simulink library "xps_library"  (Simulink 8.0)
settings: Solver=ode45  SolverMode=SingleTasking  StartTime=0.0  StopTime=10.0  RelTol=1e-3
undefined symbols (not defined in the file): sys_clk, xps_library_software_register_user_data_in
libraries: xbsIndex_r4 x867, simulink x109, dspsigops x81, casper_library_flow_control x68, xps_library x18, casper_library_misc x11
(part 2 of 10)

== system xps_library/XAUI ==
  rx_get : Inport
  rx_reset : Inport  Port=2
  tx_data : Inport  Port=3
  tx_outofband : Inport  Port=4
  tx_valid : Inport  Port=5
  Constant{1..7} (7 alike) : Constant  Value=0
  Terminator{,1..4} (5 alike) : Terminator
  convert_rx_get : xbsIndex_r4/Convert  gui_display_data_type=Fixed-point  arith_type=Boolean  n_bits=64  bin_pt=0  float_type=Single  exp_bits=8  fraction_bits=24  quantization=Truncate  overflow=Wrap  en=off  latency=0  dbl_ovrd=off  pipeline=off  block_type=convert
      settings: xl_area=[0, 0, 0, 0, 0, 0, 0]
  convert_rx_reset : xbsIndex_r4/Convert  gui_display_data_type=Fixed-point  arith_type=Boolean  n_bits=1  bin_pt=0  float_type=Single  exp_bits=8  fraction_bits=24  quantization=Truncate  overflow=Wrap  en=off  latency=0  dbl_ovrd=off  pipeline=off  block_type=convert
      settings: xl_area=[0, 0, 0, 0, 0, 0, 0]
  convert_tx_data : xbsIndex_r4/Convert  gui_display_data_type=Fixed-point  arith_type=Unsigned  n_bits=64  bin_pt=0  float_type=Single  exp_bits=8  fraction_bits=24  quantization=Truncate  overflow=Wrap  en=off  latency=0  dbl_ovrd=off  pipeline=off  block_type=convert
      settings: xl_area=[0, 0, 0, 0, 0, 0, 0]
  convert_tx_outofband : xbsIndex_r4/Convert  gui_display_data_type=Fixed-point  arith_type=Unsigned  n_bits=8  bin_pt=0  float_type=Single  exp_bits=8  fraction_bits=24  quantization=Truncate  overflow=Wrap  en=off  latency=0  dbl_ovrd=off  pipeline=off  block_type=convert
      settings: xl_area=[0, 0, 0, 0, 0, 0, 0]
  convert_tx_valid : xbsIndex_r4/Convert  gui_display_data_type=Fixed-point  arith_type=Boolean  n_bits=1  bin_pt=0  float_type=Single  exp_bits=8  fraction_bits=24  quantization=Truncate  overflow=Wrap  en=off  latency=0  dbl_ovrd=off  pipeline=off  block_type=convert
      settings: xl_area=[0, 0, 0, 0, 0, 0, 0]
  r_xaui_test_XAUI_rx_almost_full : xbsIndex_r4/Gateway In  gui_display_data_type=Fixed-point  arith_type=Boolean  n_bits=1  bin_pt=0  preci_type=Single  exp_width=8  frac_width=24  quantization=Truncate  overflow=Wrap  period=1  dbl_ovrd=off  timing_constraint=None  locs_specified=off  LOCs={}  hdl_port=on  block_type=gatewayin
      settings: infoedit="Gateway in block.  Converts inputs of type Simulink integer, double and fixed point to  Xilinx fixed point type.<P><P>Hardware notes:  In hardware these blocks become top level input ports."  xl_area=[0, 0, 0, 0, 0, 0, 0]
  r_xaui_test_XAUI_rx_data : xbsIndex_r4/Gateway In  gui_display_data_type=Fixed-point  arith_type=Unsigned  n_bits=64  bin_pt=0  preci_type=Single  exp_width=8  frac_width=24  quantization=Truncate  overflow=Wrap  period=1  dbl_ovrd=off  timing_constraint=None  locs_specified=off  LOCs={}  hdl_port=on  block_type=gatewayin
      settings: infoedit="Gateway in block.  Converts inputs of type Simulink integer, double and fixed point to  Xilinx fixed point type.<P><P>Hardware notes:  In hardware these blocks become top level input ports."  xl_area=[0, 0, 0, 0, 0, 0, 0]
  r_xaui_test_XAUI_rx_empty : xbsIndex_r4/Gateway In  gui_display_data_type=Fixed-point  arith_type=Boolean  n_bits=1  bin_pt=0  preci_type=Single  exp_width=8  frac_width=24  quantization=Truncate  overflow=Wrap  period=1  dbl_ovrd=off  timing_constraint=None  locs_specified=off  LOCs={}  hdl_port=on  block_type=gatewayin
      settings: infoedit="Gateway in block.  Converts inputs of type Simulink integer, double and fixed point to  Xilinx fixed point type.<P><P>Hardware notes:  In hardware these blocks become top level input ports."  xl_area=[0, 0, 0, 0, 0, 0, 0]
  r_xaui_test_XAUI_rx_get : xbsIndex_r4/Gateway Out  hdl_port=on  timing_constraint=None  locs_specified=off  LOCs={}  block_type=gatewayout
      settings: infoedit="Gateway out block.  Converts Xilinx fixed point inputs into ouputs of type Simulink integer, double, or fixed point.<P><P>Hardware notes:  In hardware these blocks become top level output ports or are discarded, depending on how they are configured."  xl_area=[0, 0, 0, 0, 0, 0, 0]
  r_xaui_test_XAUI_rx_linkdown : xbsIndex_r4/Gateway In  gui_display_data_type=Fixed-point  arith_type=Boolean  n_bits=1  bin_pt=0  preci_type=Single  exp_width=8  frac_width=24  quantization=Truncate  overflow=Wrap  period=1  dbl_ovrd=off  timing_constraint=None  locs_specified=off  LOCs={}  hdl_port=on  block_type=gatewayin
      settings: infoedit="Gateway in block.  Converts inputs of type Simulink integer, double and fixed point to  Xilinx fixed point type.<P><P>Hardware notes:  In hardware these blocks become top level input ports."  xl_area=[0, 0, 0, 0, 0, 0, 0]
  r_xaui_test_XAUI_rx_outofband : xbsIndex_r4/Gateway In  gui_display_data_type=Fixed-point  arith_type=Unsigned  n_bits=8  bin_pt=0  preci_type=Single  exp_width=8  frac_width=24  quantization=Truncate  overflow=Wrap  period=1  dbl_ovrd=off  timing_constraint=None  locs_specified=off  LOCs={}  hdl_port=on  block_type=gatewayin
      settings: infoedit="Gateway in block.  Converts inputs of type Simulink integer, double and fixed point to  Xilinx fixed point type.<P><P>Hardware notes:  In hardware these blocks become top level input ports."  xl_area=[0, 0, 0, 0, 0, 0, 0]
  r_xaui_test_XAUI_rx_reset : xbsIndex_r4/Gateway Out  hdl_port=on  timing_constraint=None  locs_specified=off  LOCs={}  block_type=gatewayout
      settings: infoedit="Gateway out block.  Converts Xilinx fixed point inputs into ouputs of type Simulink integer, double, or fixed point.<P><P>Hardware notes:  In hardware these blocks become top level output ports or are discarded, depending on how they are configured."  xl_area=[0, 0, 0, 0, 0, 0, 0]
  r_xaui_test_XAUI_rx_valid : xbsIndex_r4/Gateway In  gui_display_data_type=Fixed-point  arith_type=Boolean  n_bits=1  bin_pt=0  preci_type=Single  exp_width=8  frac_width=24  quantization=Truncate  overflow=Wrap  period=1  dbl_ovrd=off  timing_constraint=None  locs_specified=off  LOCs={}  hdl_port=on  block_type=gatewayin
      settings: infoedit="Gateway in block.  Converts inputs of type Simulink integer, double and fixed point to  Xilinx fixed point type.<P><P>Hardware notes:  In hardware these blocks become top level input ports."  xl_area=[0, 0, 0, 0, 0, 0, 0]
  r_xaui_test_XAUI_tx_data : xbsIndex_r4/Gateway Out  hdl_port=on  timing_constraint=None  locs_specified=off  LOCs={}  block_type=gatewayout
      settings: infoedit="Gateway out block.  Converts Xilinx fixed point inputs into ouputs of type Simulink integer, double, or fixed point.<P><P>Hardware notes:  In hardware these blocks become top level output ports or are discarded, depending on how they are configured."  xl_area=[0, 0, 0, 0, 0, 0, 0]
  r_xaui_test_XAUI_tx_full : xbsIndex_r4/Gateway In  gui_display_data_type=Fixed-point  arith_type=Boolean  n_bits=1  bin_pt=0  preci_type=Single  exp_width=8  frac_width=24  quantization=Truncate  overflow=Wrap  period=1  dbl_ovrd=off  timing_constraint=None  locs_specified=off  LOCs={}  hdl_port=on  block_type=gatewayin
      settings: infoedit="Gateway in block.  Converts inputs of type Simulink integer, double and fixed point to  Xilinx fixed point type.<P><P>Hardware notes:  In hardware these blocks become top level input ports."  xl_area=[0, 0, 0, 0, 0, 0, 0]
  r_xaui_test_XAUI_tx_outofband : xbsIndex_r4/Gateway Out  hdl_port=on  timing_constraint=None  locs_specified=off  LOCs={}  block_type=gatewayout
      settings: infoedit="Gateway out block.  Converts Xilinx fixed point inputs into ouputs of type Simulink integer, double, or fixed point.<P><P>Hardware notes:  In hardware these blocks become top level output ports or are discarded, depending on how they are configured."  xl_area=[0, 0, 0, 0, 0, 0, 0]
  r_xaui_test_XAUI_tx_valid : xbsIndex_r4/Gateway Out  hdl_port=on  timing_constraint=None  locs_specified=off  LOCs={}  block_type=gatewayout
      settings: infoedit="Gateway out block.  Converts Xilinx fixed point inputs into ouputs of type Simulink integer, double, or fixed point.<P><P>Hardware notes:  In hardware these blocks become top level output ports or are discarded, depending on how they are configured."  xl_area=[0, 0, 0, 0, 0, 0, 0]
  rx_data : Outport
  rx_outofband : Outport  Port=2
  rx_empty : Outport  Port=3
  rx_valid : Outport  Port=4
  rx_linkdown : Outport  Port=5
  tx_full : Outport  Port=6
  rx_almost_full : Outport  Port=7
  wires:
  rx_get/1 -> convert_rx_get/1
  convert_rx_get/1 -> r_xaui_test_XAUI_rx_get/1
  rx_reset/1 -> convert_rx_reset/1
  convert_rx_reset/1 -> r_xaui_test_XAUI_rx_reset/1
  r_xaui_test_XAUI_rx_data/1 -> rx_data/1
  r_xaui_test_XAUI_rx_outofband/1 -> rx_outofband/1
  r_xaui_test_XAUI_rx_empty/1 -> rx_empty/1
  r_xaui_test_XAUI_rx_linkdown/1 -> rx_linkdown/1
  tx_data/1 -> convert_tx_data/1
  convert_tx_data/1 -> r_xaui_test_XAUI_tx_data/1
  tx_outofband/1 -> convert_tx_outofband/1
  convert_tx_outofband/1 -> r_xaui_test_XAUI_tx_outofband/1
  tx_valid/1 -> convert_tx_valid/1
  convert_tx_valid/1 -> r_xaui_test_XAUI_tx_valid/1
  r_xaui_test_XAUI_tx_full/1 -> tx_full/1
  r_xaui_test_XAUI_tx_data/1 -> Terminator/1
  r_xaui_test_XAUI_tx_outofband/1 -> Terminator1/1
  r_xaui_test_XAUI_tx_valid/1 -> Terminator2/1
  Constant2/1 -> r_xaui_test_XAUI_tx_full/1
  Constant3/1 -> r_xaui_test_XAUI_rx_linkdown/1
  Constant4/1 -> r_xaui_test_XAUI_rx_empty/1
  Constant5/1 -> r_xaui_test_XAUI_rx_outofband/1
  Constant6/1 -> r_xaui_test_XAUI_rx_data/1
  r_xaui_test_XAUI_rx_get/1 -> Terminator3/1
  r_xaui_test_XAUI_rx_reset/1 -> Terminator4/1
  Constant7/1 -> r_xaui_test_XAUI_rx_valid/1
  r_xaui_test_XAUI_rx_valid/1 -> rx_valid/1
  r_xaui_test_XAUI_rx_almost_full/1 -> rx_almost_full/1
  Constant1/1 -> r_xaui_test_XAUI_rx_almost_full/1

== system xps_library/XSG core config ==

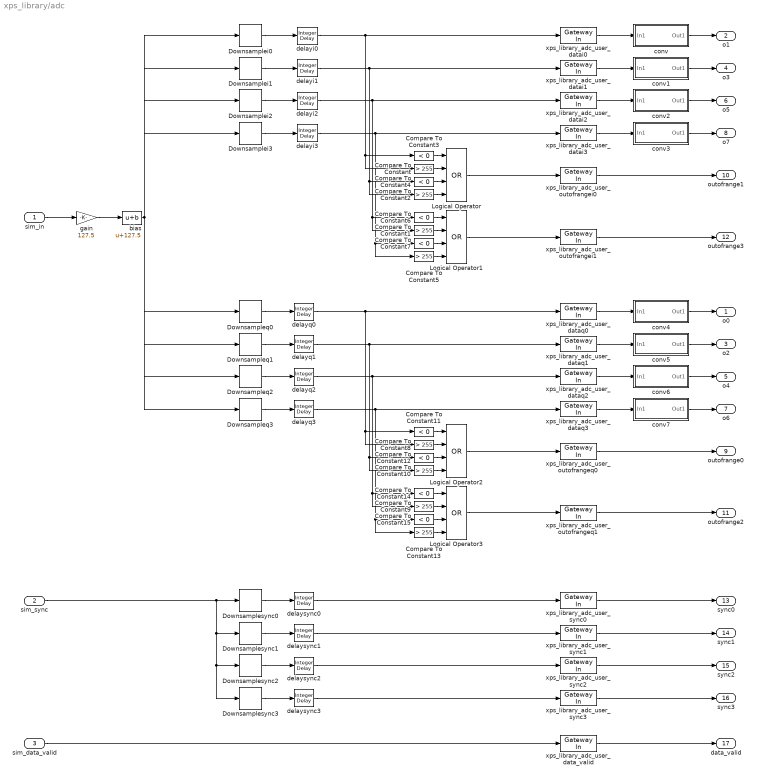
== system xps_library/adc ==
  sim_in : Inport  SampleTime=sample_period/8
  sim_sync : Inport  Port=2  SampleTime=sample_period/8
  sim_data_valid : Inport  Port=3  SampleTime=sample_period/4
  Compare To Constant{,1..2,5,8..10,13} (8 alike) : simulink/Logic and Bit Operations/Compare To Constant  relop=>  const=255  LogicOutDataTypeMode=boolean  ZeroCross=off
  Compare To Constant{3..4,6..7,11..12,14..15} (8 alike) : simulink/Logic and Bit Operations/Compare To Constant  relop=<  const=0  LogicOutDataTypeMode=boolean  ZeroCross=off
  Downsamplei0 : dspsigops/Downsample  N=8  phase=1  smode=Allow multirate  fmode=Maintain input frame size  ic=0
  Downsamplei1 : dspsigops/Downsample  N=8  phase=3  smode=Allow multirate  fmode=Maintain input frame size  ic=0
  Downsamplei2 : dspsigops/Downsample  N=8  phase=5  smode=Allow multirate  fmode=Maintain input frame size  ic=0
  Downsamplei3 : dspsigops/Downsample  N=8  phase=7  smode=Allow multirate  fmode=Maintain input frame size  ic=0
  Downsampleq0 : dspsigops/Downsample  N=8  phase=0  smode=Allow multirate  fmode=Maintain input frame size  ic=0
  Downsampleq1 : dspsigops/Downsample  N=8  phase=2  smode=Allow multirate  fmode=Maintain input frame size  ic=0
  Downsampleq2 : dspsigops/Downsample  N=8  phase=4  smode=Allow multirate  fmode=Maintain input frame size  ic=0
  Downsampleq3 : dspsigops/Downsample  N=8  phase=6  smode=Allow multirate  fmode=Maintain input frame size  ic=0
  Downsamplesync0 : dspsigops/Downsample  N=8  phase=0  smode=Allow multirate  fmode=Maintain input frame size  ic=0
  Downsamplesync1 : dspsigops/Downsample  N=8  phase=2  smode=Allow multirate  fmode=Maintain input frame size  ic=0
  Downsamplesync2 : dspsigops/Downsample  N=8  phase=4  smode=Allow multirate  fmode=Maintain input frame size  ic=0
  Downsamplesync3 : dspsigops/Downsample  N=8  phase=6  smode=Allow multirate  fmode=Maintain input frame size  ic=0
  Logical Operator{,1..3} (4 alike) : Logic  Operator=OR  Inputs=4  AllPortsSameDT=off  OutDataTypeStr=boolean
  bias : Bias  Bias=127.5  SaturateOnIntegerOverflow=on
  conv : Subsystem
  conv1 : Subsystem
  conv2 : Subsystem
  conv3 : Subsystem
  conv4 : Subsystem
  conv5 : Subsystem
  conv6 : Subsystem
  conv7 : Subsystem
  delayi{0..3} (4 alike) : simulink/Discrete/Integer Delay  NumDelays=1  vinit=0.0  samptime=-1
  delayq0 : simulink/Discrete/Integer Delay  NumDelays=2  vinit=0.0  samptime=-1
  delayq1 : simulink/Discrete/Integer Delay  NumDelays=1  vinit=0.0  samptime=-1
  delayq2 : simulink/Discrete/Integer Delay  NumDelays=1  vinit=0.0  samptime=-1
  delayq3 : simulink/Discrete/Integer Delay  NumDelays=1  vinit=0.0  samptime=-1
  delaysync0 : simulink/Discrete/Integer Delay  NumDelays=2  vinit=0.0  samptime=-1
  delaysync1 : simulink/Discrete/Integer Delay  NumDelays=1  vinit=0.0  samptime=-1
  delaysync2 : simulink/Discrete/Integer Delay  NumDelays=1  vinit=0.0  samptime=-1
  delaysync3 : simulink/Discrete/Integer Delay  NumDelays=1  vinit=0.0  samptime=-1
  gain : Gain  Gain=127.5  SaturateOnIntegerOverflow=on  OutDataTypeStr=Inherit: Same as input  ParamDataTypeStr=Inherit: Same as input
  xps_library_adc_user_data_valid : xbsIndex_r4/Gateway In  gui_display_data_type=Fixed-point  arith_type=Boolean  n_bits=8  bin_pt=0  preci_type=Single  exp_width=8  frac_width=24  quantization="Round  (unbiased: +/- Inf)"  overflow=Saturate  period=sample_period  dbl_ovrd=off  timing_constraint=None  locs_specified=off  LOCs={}  hdl_port=on  block_type=gatewayin
      settings: infoedit="Gateway in block.  Converts inputs of type Simulink integer, double and fixed point to  Xilinx fixed point type.<P><P>Hardware notes:  In hardware these blocks become top level input ports."  xl_area=[0 0 0 0 8 0 0]  block_version=8.2.02
  xps_library_adc_user_datai{0..3} (4 alike) : xbsIndex_r4/Gateway In  gui_display_data_type=Fixed-point  arith_type=Unsigned  n_bits=8  bin_pt=0  preci_type=Single  exp_width=8  frac_width=24  quantization="Round  (unbiased: +/- Inf)"  overflow=Saturate  period=sample_period  dbl_ovrd=off  timing_constraint=None  locs_specified=off  LOCs={}  hdl_port=on  block_type=gatewayin
      settings: infoedit="Gateway in block.  Converts inputs of type Simulink integer, double and fixed point to  Xilinx fixed point type.<P><P>Hardware notes:  In hardware these blocks become top level input ports."  xl_area=[0 0 0 0 8 0 0]  block_version=8.2.02
  xps_library_adc_user_dataq{0..3} (4 alike) : xbsIndex_r4/Gateway In  gui_display_data_type=Fixed-point  arith_type=Unsigned  n_bits=8  bin_pt=0  preci_type=Single  exp_width=8  frac_width=24  quantization="Round  (unbiased: +/- Inf)"  overflow=Saturate  period=sample_period  dbl_ovrd=off  timing_constraint=None  locs_specified=off  LOCs={}  hdl_port=on  block_type=gatewayin
      settings: infoedit="Gateway in block.  Converts inputs of type Simulink integer, double and fixed point to  Xilinx fixed point type.<P><P>Hardware notes:  In hardware these blocks become top level input ports."  xl_area=[0 0 0 0 8 0 0]  block_version=8.2.02
  xps_library_adc_user_outofrangei0 : xbsIndex_r4/Gateway In  gui_display_data_type=Fixed-point  arith_type=Boolean  n_bits=8  bin_pt=0  preci_type=Single  exp_width=8  frac_width=24  quantization="Round  (unbiased: +/- Inf)"  overflow=Saturate  period=sample_period  dbl_ovrd=off  timing_constraint=None  locs_specified=off  LOCs={}  hdl_port=on  block_type=gatewayin
      settings: infoedit="Gateway in block.  Converts inputs of type Simulink integer, double and fixed point to  Xilinx fixed point type.<P><P>Hardware notes:  In hardware these blocks become top level input ports."  xl_area=[0 0 0 0 8 0 0]  block_version=8.2.02
  xps_library_adc_user_outofrangei1 : xbsIndex_r4/Gateway In  gui_display_data_type=Fixed-point  arith_type=Boolean  n_bits=8  bin_pt=0  preci_type=Single  exp_width=8  frac_width=24  quantization="Round  (unbiased: +/- Inf)"  overflow=Saturate  period=sample_period  dbl_ovrd=off  timing_constraint=None  locs_specified=off  LOCs={}  hdl_port=on  block_type=gatewayin
      settings: infoedit="Gateway in block.  Converts inputs of type Simulink integer, double and fixed point to  Xilinx fixed point type.<P><P>Hardware notes:  In hardware these blocks become top level input ports."  xl_area=[0 0 0 0 8 0 0]  block_version=8.2.02
  xps_library_adc_user_outofrangeq0 : xbsIndex_r4/Gateway In  gui_display_data_type=Fixed-point  arith_type=Boolean  n_bits=8  bin_pt=0  preci_type=Single  exp_width=8  frac_width=24  quantization="Round  (unbiased: +/- Inf)"  overflow=Saturate  period=sample_period  dbl_ovrd=off  timing_constraint=None  locs_specified=off  LOCs={}  hdl_port=on  block_type=gatewayin
      settings: infoedit="Gateway in block.  Converts inputs of type Simulink integer, double and fixed point to  Xilinx fixed point type.<P><P>Hardware notes:  In hardware these blocks become top level input ports."  xl_area=[0 0 0 0 8 0 0]  block_version=8.2.02
  xps_library_adc_user_outofrangeq1 : xbsIndex_r4/Gateway In  gui_display_data_type=Fixed-point  arith_type=Boolean  n_bits=8  bin_pt=0  preci_type=Single  exp_width=8  frac_width=24  quantization="Round  (unbiased: +/- Inf)"  overflow=Saturate  period=sample_period  dbl_ovrd=off  timing_constraint=None  locs_specified=off  LOCs={}  hdl_port=on  block_type=gatewayin
      settings: infoedit="Gateway in block.  Converts inputs of type Simulink integer, double and fixed point to  Xilinx fixed point type.<P><P>Hardware notes:  In hardware these blocks become top level input ports."  xl_area=[0 0 0 0 8 0 0]  block_version=8.2.02
  xps_library_adc_user_sync{0..3} (4 alike) : xbsIndex_r4/Gateway In  gui_display_data_type=Fixed-point  arith_type=Boolean  n_bits=8  bin_pt=0  preci_type=Single  exp_width=8  frac_width=24  quantization="Round  (unbiased: +/- Inf)"  overflow=Saturate  period=sample_period  dbl_ovrd=off  timing_constraint=None  locs_specified=off  LOCs={}  hdl_port=on  block_type=gatewayin
      settings: infoedit="Gateway in block.  Converts inputs of type Simulink integer, double and fixed point to  Xilinx fixed point type.<P><P>Hardware notes:  In hardware these blocks become top level input ports."  xl_area=[0 0 0 0 8 0 0]  block_version=8.2.02
  o0 : Outport
  o1 : Outport  Port=2
  o2 : Outport  Port=3
  o3 : Outport  Port=4
  o4 : Outport  Port=5
  o5 : Outport  Port=6
  o6 : Outport  Port=7
  o7 : Outport  Port=8
  outofrange0 : Outport  Port=9
  outofrange1 : Outport  Port=10
  outofrange2 : Outport  Port=11
  outofrange3 : Outport  Port=12
  sync0 : Outport  Port=13
  sync1 : Outport  Port=14
  sync2 : Outport  Port=15
  sync3 : Outport  Port=16
  data_valid : Outport  Port=17
  wires:
  delaysync1/1 -> xps_library_adc_user_sync1/1
  delayq3/1 -> xps_library_adc_user_dataq3/1, Compare To Constant15/1, Compare To Constant13/1
  delayq2/1 -> xps_library_adc_user_dataq2/1, Compare To Constant14/1, Compare To Constant9/1
  delayq1/1 -> xps_library_adc_user_dataq1/1, Compare To Constant12/1, Compare To Constant10/1
  delayi3/1 -> xps_library_adc_user_datai3/1, Compare To Constant7/1, Compare To Constant5/1
  delayi2/1 -> xps_library_adc_user_datai2/1, Compare To Constant6/1, Compare To Constant1/1
  delayi1/1 -> xps_library_adc_user_datai1/1, Compare To Constant2/1, Compare To Constant4/1
  Downsamplei0/1 -> delayi0/1
  conv7/1(Out1) -> o6/1
  xps_library_adc_user_dataq3/1 -> conv7/1(In1)
  conv6/1(Out1) -> o4/1
  xps_library_adc_user_dataq2/1 -> conv6/1(In1)
  conv5/1(Out1) -> o2/1
  xps_library_adc_user_dataq1/1 -> conv5/1(In1)
  conv4/1(Out1) -> o0/1
  xps_library_adc_user_dataq0/1 -> conv4/1(In1)
  conv3/1(Out1) -> o7/1
  conv2/1(Out1) -> o5/1
  conv1/1(Out1) -> o3/1
  conv/1(Out1) -> o1/1
  xps_library_adc_user_sync0/1 -> sync0/1
  xps_library_adc_user_outofrangei0/1 -> outofrange1/1
  xps_library_adc_user_datai3/1 -> conv3/1(In1)
  xps_library_adc_user_datai2/1 -> conv2/1(In1)
  xps_library_adc_user_datai1/1 -> conv1/1(In1)
  Downsampleq3/1 -> delayq3/1
  Downsampleq2/1 -> delayq2/1
  Downsampleq1/1 -> delayq1/1
  Downsamplei3/1 -> delayi3/1
  Downsamplei2/1 -> delayi2/1
  Downsamplei1/1 -> delayi1/1
  delayi0/1 -> xps_library_adc_user_datai0/1, Compare To Constant/1, Compare To Constant3/1
  Downsampleq0/1 -> delayq0/1
  delayq0/1 -> xps_library_adc_user_dataq0/1, Compare To Constant11/1, Compare To Constant8/1
  xps_library_adc_user_outofrangei1/1 -> outofrange3/1
  Compare To Constant3/1 -> Logical Operator/1
  Compare To Constant/1 -> Logical Operator/2
  Compare To Constant4/1 -> Logical Operator/3
  Compare To Constant2/1 -> Logical Operator/4
  Logical Operator/1 -> xps_library_adc_user_outofrangei0/1
  Compare To Constant6/1 -> Logical Operator1/1
  Compare To Constant1/1 -> Logical Operator1/2
  Compare To Constant7/1 -> Logical Operator1/3
  Compare To Constant5/1 -> Logical Operator1/4
  Logical Operator1/1 -> xps_library_adc_user_outofrangei1/1
  xps_library_adc_user_outofrangeq0/1 -> outofrange0/1
  xps_library_adc_user_outofrangeq1/1 -> outofrange2/1
  Compare To Constant11/1 -> Logical Operator2/1
  Compare To Constant8/1 -> Logical Operator2/2
  Compare To Constant12/1 -> Logical Operator2/3
  Compare To Constant10/1 -> Logical Operator2/4
  Logical Operator2/1 -> xps_library_adc_user_outofrangeq0/1
  Compare To Constant14/1 -> Logical Operator3/1
  Compare To Constant9/1 -> Logical Operator3/2
  Compare To Constant15/1 -> Logical Operator3/3
  Compare To Constant13/1 -> Logical Operator3/4
  Logical Operator3/1 -> xps_library_adc_user_outofrangeq1/1
  sim_sync/1 -> Downsamplesync0/1, Downsamplesync1/1, Downsamplesync2/1, Downsamplesync3/1
  Downsamplesync0/1 -> delaysync0/1
  Downsamplesync1/1 -> delaysync1/1
  delaysync0/1 -> xps_library_adc_user_sync0/1
  xps_library_adc_user_sync1/1 -> sync1/1
  Downsamplesync2/1 -> delaysync2/1
  Downsamplesync3/1 -> delaysync3/1
  delaysync2/1 -> xps_library_adc_user_sync2/1
  delaysync3/1 -> xps_library_adc_user_sync3/1
  xps_library_adc_user_sync2/1 -> sync2/1
  xps_library_adc_user_sync3/1 -> sync3/1
  xps_library_adc_user_data_valid/1 -> data_valid/1
  sim_data_valid/1 -> xps_library_adc_user_data_valid/1
  xps_library_adc_user_datai0/1 -> conv/1(In1)
  sim_in/1 -> gain/1
  gain/1 -> bias/1
  bias/1 -> Downsamplei0/1, Downsamplei1/1, Downsamplei2/1, Downsamplei3/1, Downsampleq0/1, Downsampleq1/1, Downsampleq2/1, Downsampleq3/1

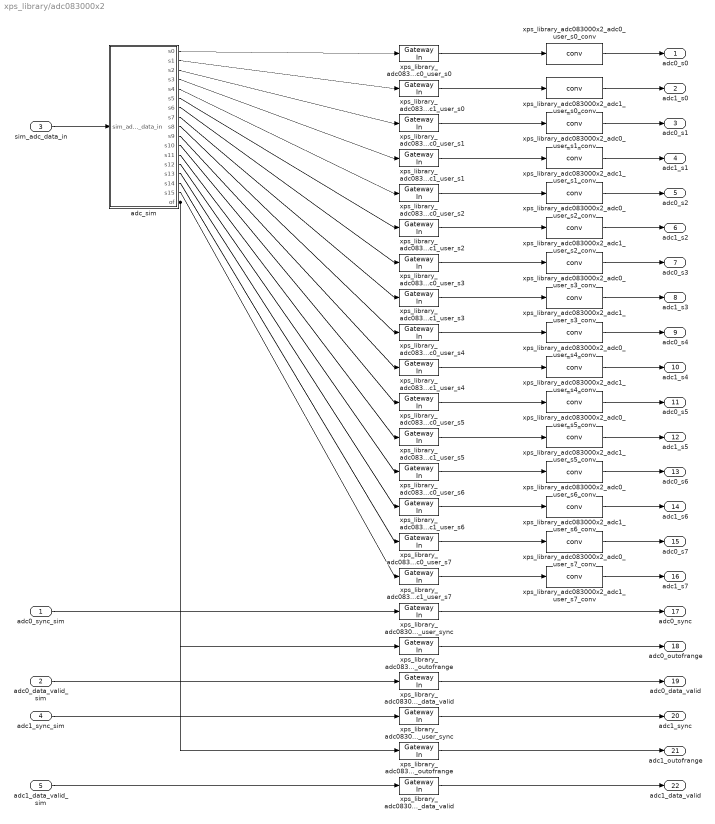
== system xps_library/adc083000x2 ==
  adc0_sync_sim : Inport
  adc0_data_valid_sim : Inport  Port=2
  sim_adc_data_in : Inport  Port=3
  adc1_sync_sim : Inport  Port=4
  adc1_data_valid_sim : Inport  Port=5
  adc_sim : Subsystem  AncestorBlock=xps_library/ADCs/adc_sim  mask(adc_sim){nStreams=16, bit_width=8}
      mask prompts: nStreams "Number of Output Streams"; bit_width "Sample Bit Width"
      mask help:
      | This block simulates the behavior of a demuxed ADC, which takes
      | as input a waveform and returns digital samples in parallel at
      | a slower rate.
      |
      | This block is used to simulate the behavior
      mask init:
      | adc_sim_init(gcb, ...
      |     'nStreams', nStreams, ...
      |     'bit_width', bit_width);
  xps_library_adc083000x2_adc0_user_data_valid : xbsIndex_r4/Gateway In  gui_display_data_type=Fixed-point  arith_type=Unsigned  n_bits=1  bin_pt=0  preci_type=Single  exp_width=8  frac_width=24  quantization="Round  (unbiased: +/- Inf)"  overflow=Saturate  period=1  dbl_ovrd=off  timing_constraint=None  locs_specified=off  LOCs={}  hdl_port=on  block_type=gatewayin
  xps_library_adc083000x2_adc0_user_outofrange : xbsIndex_r4/Gateway In  gui_display_data_type=Fixed-point  arith_type=Unsigned  n_bits=4  bin_pt=0  preci_type=Single  exp_width=8  frac_width=24  quantization="Round  (unbiased: +/- Inf)"  overflow=Saturate  period=1  dbl_ovrd=off  timing_constraint=None  locs_specified=off  LOCs={}  hdl_port=on  block_type=gatewayin
  xps_library_adc083000x2_adc0_user_s{0..7} (8 alike) : xbsIndex_r4/Gateway In  gui_display_data_type=Fixed-point  arith_type=Unsigned  n_bits=8  bin_pt=0  preci_type=Single  exp_width=8  frac_width=24  quantization="Round  (unbiased: +/- Inf)"  overflow=Saturate  period=1  dbl_ovrd=off  timing_constraint=None  locs_specified=off  LOCs={}  hdl_port=on  block_type=gatewayin
  xps_library_adc083000x2_adc0_user_s0_conv : xps_library/ADCs/conv  bit_width=8
  xps_library_adc083000x2_adc0_user_s1_conv : xps_library/ADCs/conv  bit_width=8
  xps_library_adc083000x2_adc0_user_s2_conv : xps_library/ADCs/conv  bit_width=8
  xps_library_adc083000x2_adc0_user_s3_conv : xps_library/ADCs/conv  bit_width=8
  xps_library_adc083000x2_adc0_user_s4_conv : xps_library/ADCs/conv  bit_width=8
  xps_library_adc083000x2_adc0_user_s5_conv : xps_library/ADCs/conv  bit_width=8
  xps_library_adc083000x2_adc0_user_s6_conv : xps_library/ADCs/conv  bit_width=8
  xps_library_adc083000x2_adc0_user_s7_conv : xps_library/ADCs/conv  bit_width=8
  xps_library_adc083000x2_adc0_user_sync : xbsIndex_r4/Gateway In  gui_display_data_type=Fixed-point  arith_type=Unsigned  n_bits=4  bin_pt=0  preci_type=Single  exp_width=8  frac_width=24  quantization="Round  (unbiased: +/- Inf)"  overflow=Saturate  period=1  dbl_ovrd=off  timing_constraint=None  locs_specified=off  LOCs={}  hdl_port=on  block_type=gatewayin
  xps_library_adc083000x2_adc1_user_data_valid : xbsIndex_r4/Gateway In  gui_display_data_type=Fixed-point  arith_type=Unsigned  n_bits=1  bin_pt=0  preci_type=Single  exp_width=8  frac_width=24  quantization="Round  (unbiased: +/- Inf)"  overflow=Saturate  period=1  dbl_ovrd=off  timing_constraint=None  locs_specified=off  LOCs={}  hdl_port=on  block_type=gatewayin  OutDataTypeMode=boolean
  xps_library_adc083000x2_adc1_user_outofrange : xbsIndex_r4/Gateway In  gui_display_data_type=Fixed-point  arith_type=Unsigned  n_bits=4  bin_pt=0  preci_type=Single  exp_width=8  frac_width=24  quantization="Round  (unbiased: +/- Inf)"  overflow=Saturate  period=1  dbl_ovrd=off  timing_constraint=None  locs_specified=off  LOCs={}  hdl_port=on  block_type=gatewayin
  xps_library_adc083000x2_adc1_user_s{0..7} (8 alike) : xbsIndex_r4/Gateway In  gui_display_data_type=Fixed-point  arith_type=Unsigned  n_bits=8  bin_pt=0  preci_type=Single  exp_width=8  frac_width=24  quantization="Round  (unbiased: +/- Inf)"  overflow=Saturate  period=1  dbl_ovrd=off  timing_constraint=None  locs_specified=off  LOCs={}  hdl_port=on  block_type=gatewayin
  xps_library_adc083000x2_adc1_user_s0_conv : xps_library/ADCs/conv  bit_width=8
  xps_library_adc083000x2_adc1_user_s1_conv : xps_library/ADCs/conv  bit_width=8
  xps_library_adc083000x2_adc1_user_s2_conv : xps_library/ADCs/conv  bit_width=8
  xps_library_adc083000x2_adc1_user_s3_conv : xps_library/ADCs/conv  bit_width=8
  xps_library_adc083000x2_adc1_user_s4_conv : xps_library/ADCs/conv  bit_width=8
  xps_library_adc083000x2_adc1_user_s5_conv : xps_library/ADCs/conv  bit_width=8
  xps_library_adc083000x2_adc1_user_s6_conv : xps_library/ADCs/conv  bit_width=8
  xps_library_adc083000x2_adc1_user_s7_conv : xps_library/ADCs/conv  bit_width=8
  xps_library_adc083000x2_adc1_user_sync : xbsIndex_r4/Gateway In  gui_display_data_type=Fixed-point  arith_type=Unsigned  n_bits=4  bin_pt=0  preci_type=Single  exp_width=8  frac_width=24  quantization="Round  (unbiased: +/- Inf)"  overflow=Saturate  period=1  dbl_ovrd=off  timing_constraint=None  locs_specified=off  LOCs={}  hdl_port=on  block_type=gatewayin
  adc0_s0 : Outport
  adc1_s0 : Outport  Port=2
  adc0_s1 : Outport  Port=3
  adc1_s1 : Outport  Port=4
  adc0_s2 : Outport  Port=5
  adc1_s2 : Outport  Port=6
  adc0_s3 : Outport  Port=7
  adc1_s3 : Outport  Port=8
  adc0_s4 : Outport  Port=9
  adc1_s4 : Outport  Port=10
  adc0_s5 : Outport  Port=11
  adc1_s5 : Outport  Port=12
  adc0_s6 : Outport  Port=13
  adc1_s6 : Outport  Port=14
  adc0_s7 : Outport  Port=15
  adc1_s7 : Outport  Port=16
  adc0_sync : Outport  Port=17
  adc0_outofrange : Outport  Port=18
  adc0_data_valid : Outport  Port=19
  adc1_sync : Outport  Port=20
  adc1_outofrange : Outport  Port=21
  adc1_data_valid : Outport  Port=22
  wires:
  sim_adc_data_in/1 -> adc_sim/1(sim_adc_data_in)
  adc_sim/1(s0) -> xps_library_adc083000x2_adc0_user_s0/1
  xps_library_adc083000x2_adc0_user_s0/1 -> xps_library_adc083000x2_adc0_user_s0_conv/1
  xps_library_adc083000x2_adc0_user_s0_conv/1 -> adc0_s0/1
  adc_sim/2(s1) -> xps_library_adc083000x2_adc1_user_s0/1
  xps_library_adc083000x2_adc1_user_s0/1 -> xps_library_adc083000x2_adc1_user_s0_conv/1
  xps_library_adc083000x2_adc1_user_s0_conv/1 -> adc1_s0/1
  adc_sim/3(s2) -> xps_library_adc083000x2_adc0_user_s1/1
  xps_library_adc083000x2_adc0_user_s1/1 -> xps_library_adc083000x2_adc0_user_s1_conv/1
  xps_library_adc083000x2_adc0_user_s1_conv/1 -> adc0_s1/1
  adc_sim/4(s3) -> xps_library_adc083000x2_adc1_user_s1/1
  xps_library_adc083000x2_adc1_user_s1/1 -> xps_library_adc083000x2_adc1_user_s1_conv/1
  xps_library_adc083000x2_adc1_user_s1_conv/1 -> adc1_s1/1
  adc_sim/5(s4) -> xps_library_adc083000x2_adc0_user_s2/1
  xps_library_adc083000x2_adc0_user_s2/1 -> xps_library_adc083000x2_adc0_user_s2_conv/1
  xps_library_adc083000x2_adc0_user_s2_conv/1 -> adc0_s2/1
  adc_sim/6(s5) -> xps_library_adc083000x2_adc1_user_s2/1
  xps_library_adc083000x2_adc1_user_s2/1 -> xps_library_adc083000x2_adc1_user_s2_conv/1
  xps_library_adc083000x2_adc1_user_s2_conv/1 -> adc1_s2/1
  adc_sim/7(s6) -> xps_library_adc083000x2_adc0_user_s3/1
  xps_library_adc083000x2_adc0_user_s3/1 -> xps_library_adc083000x2_adc0_user_s3_conv/1
  xps_library_adc083000x2_adc0_user_s3_conv/1 -> adc0_s3/1
  adc_sim/8(s7) -> xps_library_adc083000x2_adc1_user_s3/1
  xps_library_adc083000x2_adc1_user_s3/1 -> xps_library_adc083000x2_adc1_user_s3_conv/1
  xps_library_adc083000x2_adc1_user_s3_conv/1 -> adc1_s3/1
  adc_sim/9(s8) -> xps_library_adc083000x2_adc0_user_s4/1
  xps_library_adc083000x2_adc0_user_s4/1 -> xps_library_adc083000x2_adc0_user_s4_conv/1
  xps_library_adc083000x2_adc0_user_s4_conv/1 -> adc0_s4/1
  adc_sim/10(s9) -> xps_library_adc083000x2_adc1_user_s4/1
  xps_library_adc083000x2_adc1_user_s4/1 -> xps_library_adc083000x2_adc1_user_s4_conv/1
  xps_library_adc083000x2_adc1_user_s4_conv/1 -> adc1_s4/1
  adc_sim/11(s10) -> xps_library_adc083000x2_adc0_user_s5/1
  xps_library_adc083000x2_adc0_user_s5/1 -> xps_library_adc083000x2_adc0_user_s5_conv/1
  xps_library_adc083000x2_adc0_user_s5_conv/1 -> adc0_s5/1
  adc_sim/12(s11) -> xps_library_adc083000x2_adc1_user_s5/1
  xps_library_adc083000x2_adc1_user_s5/1 -> xps_library_adc083000x2_adc1_user_s5_conv/1
  xps_library_adc083000x2_adc1_user_s5_conv/1 -> adc1_s5/1
  adc_sim/13(s12) -> xps_library_adc083000x2_adc0_user_s6/1
  xps_library_adc083000x2_adc0_user_s6/1 -> xps_library_adc083000x2_adc0_user_s6_conv/1
  xps_library_adc083000x2_adc0_user_s6_conv/1 -> adc0_s6/1
  adc_sim/14(s13) -> xps_library_adc083000x2_adc1_user_s6/1
  xps_library_adc083000x2_adc1_user_s6/1 -> xps_library_adc083000x2_adc1_user_s6_conv/1
  xps_library_adc083000x2_adc1_user_s6_conv/1 -> adc1_s6/1
  adc_sim/15(s14) -> xps_library_adc083000x2_adc0_user_s7/1
  xps_library_adc083000x2_adc0_user_s7/1 -> xps_library_adc083000x2_adc0_user_s7_conv/1
  xps_library_adc083000x2_adc0_user_s7_conv/1 -> adc0_s7/1
  adc_sim/16(s15) -> xps_library_adc083000x2_adc1_user_s7/1
  xps_library_adc083000x2_adc1_user_s7/1 -> xps_library_adc083000x2_adc1_user_s7_conv/1
  xps_library_adc083000x2_adc1_user_s7_conv/1 -> adc1_s7/1
  adc0_sync_sim/1 -> xps_library_adc083000x2_adc0_user_sync/1
  xps_library_adc083000x2_adc0_user_sync/1 -> adc0_sync/1
  adc_sim/17(of) -> xps_library_adc083000x2_adc0_user_outofrange/1, xps_library_adc083000x2_adc1_user_outofrange/1
  xps_library_adc083000x2_adc0_user_outofrange/1 -> adc0_outofrange/1
  adc0_data_valid_sim/1 -> xps_library_adc083000x2_adc0_user_data_valid/1
  xps_library_adc083000x2_adc0_user_data_valid/1 -> adc0_data_valid/1
  adc1_sync_sim/1 -> xps_library_adc083000x2_adc1_user_sync/1
  xps_library_adc083000x2_adc1_user_sync/1 -> adc1_sync/1
  xps_library_adc083000x2_adc1_user_outofrange/1 -> adc1_outofrange/1
  adc1_data_valid_sim/1 -> xps_library_adc083000x2_adc1_user_data_valid/1
  xps_library_adc083000x2_adc1_user_data_valid/1 -> adc1_data_valid/1

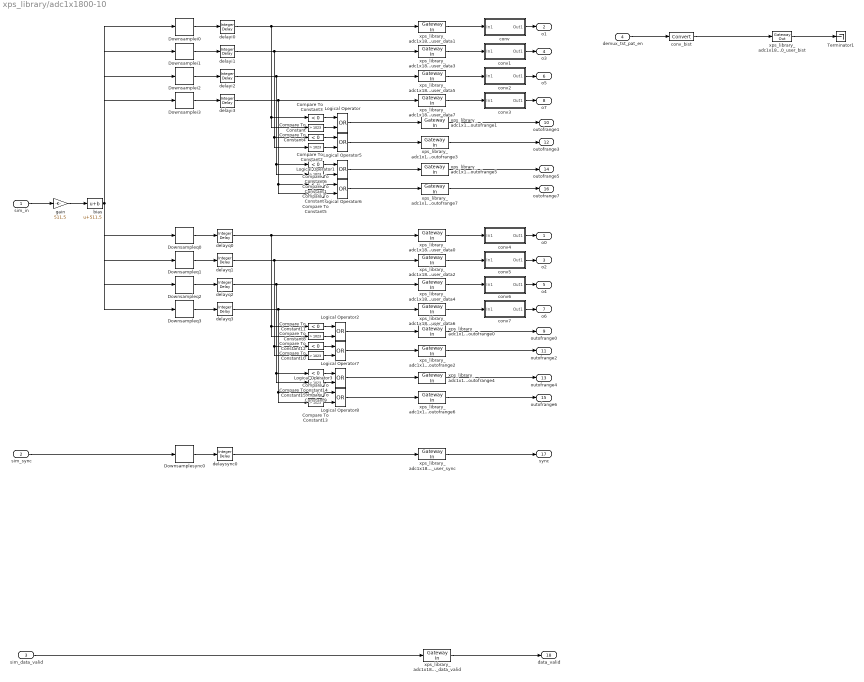
== system xps_library/adc1x1800-10 ==
  sim_in : Inport  SampleTime=sample_period/8
  sim_sync : Inport  Port=2  SampleTime=sample_period/8
  sim_data_valid : Inport  Port=3  SampleTime=sample_period/4
  demux_tst_pat_en : Inport  Port=4  SampleTime=sample_period/8
  Compare To Constant{,1..2,5,8..10,13} (8 alike) : simulink/Logic and Bit Operations/Compare To Constant  relop=>  const=1023  LogicOutDataTypeMode=boolean  ZeroCross=off
  Compare To Constant{3..4,6..7,11..12,14..15} (8 alike) : simulink/Logic and Bit Operations/Compare To Constant  relop=<  const=0  LogicOutDataTypeMode=boolean  ZeroCross=off
  Downsamplei0 : dspsigops/Downsample  N=8  phase=1  smode=Force single rate  fmode=Maintain input frame rate  ic=0
  Downsamplei1 : dspsigops/Downsample  N=8  phase=3  smode=Force single rate  fmode=Maintain input frame rate  ic=0
  Downsamplei2 : dspsigops/Downsample  N=8  phase=5  smode=Force single rate  fmode=Maintain input frame rate  ic=0
  Downsamplei3 : dspsigops/Downsample  N=8  phase=7  smode=Force single rate  fmode=Maintain input frame rate  ic=0
  Downsampleq0 : dspsigops/Downsample  N=8  phase=0  smode=Force single rate  fmode=Maintain input frame rate  ic=0
  Downsampleq1 : dspsigops/Downsample  N=8  phase=2  smode=Force single rate  fmode=Maintain input frame rate  ic=0
  Downsampleq2 : dspsigops/Downsample  N=8  phase=4  smode=Force single rate  fmode=Maintain input frame rate  ic=0
  Downsampleq3 : dspsigops/Downsample  N=8  phase=6  smode=Force single rate  fmode=Maintain input frame rate  ic=0
  Downsamplesync0 : dspsigops/Downsample  N=8  phase=0  smode=Force single rate  fmode=Maintain input frame rate  ic=0
  Logical Operator{,1..3,5..8} (8 alike) : Logic  Operator=OR  AllPortsSameDT=off  OutDataTypeStr=boolean
  Terminator1 : Terminator
  bias : Bias  Bias=511.5  SaturateOnIntegerOverflow=on
  conv : Subsystem
  conv1 : Subsystem
  conv2 : Subsystem
  conv3 : Subsystem
  conv4 : Subsystem
  conv5 : Subsystem
  conv6 : Subsystem
  conv7 : Subsystem
  conv_bist : xbsIndex_r4/Convert  gui_display_data_type=Fixed-point  arith_type=Boolean  n_bits=8  bin_pt=0  float_type=Single  exp_bits=8  fraction_bits=24  quantization=Truncate  overflow=Wrap  en=off  latency=0  dbl_ovrd=off  pipeline=off  block_type=convert
      settings: xl_area=[0, 0, 0, 0, 0, 0, 0]
  delayi{0..3} (4 alike) : simulink/Discrete/Integer Delay  NumDelays=1  vinit=0.0  samptime=-1
  delayq0 : simulink/Discrete/Integer Delay  NumDelays=2  vinit=0.0  samptime=-1
  delayq1 : simulink/Discrete/Integer Delay  NumDelays=1  vinit=0.0  samptime=-1
  delayq2 : simulink/Discrete/Integer Delay  NumDelays=1  vinit=0.0  samptime=-1
  delayq3 : simulink/Discrete/Integer Delay  NumDelays=1  vinit=0.0  samptime=-1
  delaysync0 : simulink/Discrete/Integer Delay  NumDelays=2  vinit=0.0  samptime=-1
  gain : Gain  Gain=511.5  SaturateOnIntegerOverflow=on  OutDataTypeStr=Inherit: Same as input  ParamDataTypeStr=Inherit: Same as input
  xps_library_adc1x1800_10_user_bist : xbsIndex_r4/Gateway Out  hdl_port=on  timing_constraint=None  locs_specified=off  LOCs={}  block_type=gatewayout
      settings: infoedit="Gateway out block.  Converts Xilinx fixed point inputs into ouputs of type Simulink integer, double, or fixed point.<br><br>Hardware notes:  In hardware these blocks become top level output ports or are discarded, depending on how they are configured."  block_version=11.4
  xps_library_adc1x1800_10_user_data{0..7} (8 alike) : xbsIndex_r4/Gateway In  gui_display_data_type=Fixed-point  arith_type=Unsigned  n_bits=10  bin_pt=0  preci_type=Single  exp_width=8  frac_width=24  quantization="Round  (unbiased: +/- Inf)"  overflow=Saturate  period=sample_period  dbl_ovrd=off  timing_constraint=None  locs_specified=off  LOCs={}  hdl_port=on  block_type=gatewayin
      settings: infoedit="Gateway in block.  Converts inputs of type Simulink integer, double and fixed point to  Xilinx fixed point type.<br><br>Hardware notes:  In hardware these blocks become top level input ports."  xl_area=[0 0 0 0 8 0 0]  block_version=8.2.02
  xps_library_adc1x1800_10_user_data_valid : xbsIndex_r4/Gateway In  gui_display_data_type=Fixed-point  arith_type=Boolean  n_bits=8  bin_pt=0  preci_type=Single  exp_width=8  frac_width=24  quantization="Round  (unbiased: +/- Inf)"  overflow=Saturate  period=sample_period  dbl_ovrd=off  timing_constraint=None  locs_specified=off  LOCs={}  hdl_port=on  block_type=gatewayin
      settings: infoedit="Gateway in block.  Converts inputs of type Simulink integer, double and fixed point to  Xilinx fixed point type.<P><P>Hardware notes:  In hardware these blocks become top level input ports."  xl_area=[0 0 0 0 8 0 0]  block_version=8.2.02
  xps_library_adc1x1800_10_user_outofrange{0..7} (8 alike) : xbsIndex_r4/Gateway In  gui_display_data_type=Fixed-point  arith_type=Boolean  n_bits=8  bin_pt=0  preci_type=Single  exp_width=8  frac_width=24  quantization="Round  (unbiased: +/- Inf)"  overflow=Saturate  period=sample_period  dbl_ovrd=off  timing_constraint=None  locs_specified=off  LOCs={}  hdl_port=on  block_type=gatewayin
      settings: infoedit="Gateway in block.  Converts inputs of type Simulink integer, double and fixed point to  Xilinx fixed point type.<P><P>Hardware notes:  In hardware these blocks become top level input ports."  xl_area=[0 0 0 0 8 0 0]  block_version=8.2.02
  xps_library_adc1x1800_10_user_sync : xbsIndex_r4/Gateway In  gui_display_data_type=Fixed-point  arith_type=Boolean  n_bits=8  bin_pt=0  preci_type=Single  exp_width=8  frac_width=24  quantization="Round  (unbiased: +/- Inf)"  overflow=Saturate  period=sample_period  dbl_ovrd=off  timing_constraint=None  locs_specified=off  LOCs={}  hdl_port=on  block_type=gatewayin
      settings: infoedit="Gateway in block.  Converts inputs of type Simulink integer, double and fixed point to  Xilinx fixed point type.<P><P>Hardware notes:  In hardware these blocks become top level input ports."  xl_area=[0 0 0 0 8 0 0]  block_version=8.2.02
  o0 : Outport
  o1 : Outport  Port=2
  o2 : Outport  Port=3
  o3 : Outport  Port=4
  o4 : Outport  Port=5
  o5 : Outport  Port=6
  o6 : Outport  Port=7
  o7 : Outport  Port=8
  outofrange0 : Outport  Port=9
  outofrange1 : Outport  Port=10
  outofrange2 : Outport  Port=11
  outofrange3 : Outport  Port=12
  outofrange4 : Outport  Port=13
  outofrange5 : Outport  Port=14
  outofrange6 : Outport  Port=15
  outofrange7 : Outport  Port=16
  sync : Outport  Port=17
  data_valid : Outport  Port=18
  wires:
  delayq3/1 -> xps_library_adc1x1800_10_user_data6/1, Compare To Constant15/1, Compare To Constant13/1
  delayq2/1 -> xps_library_adc1x1800_10_user_data4/1, Compare To Constant14/1, Compare To Constant9/1
  delayq1/1 -> xps_library_adc1x1800_10_user_data2/1, Compare To Constant12/1, Compare To Constant10/1
  delayi3/1 -> xps_library_adc1x1800_10_user_data7/1, Compare To Constant7/1, Compare To Constant5/1
  delayi2/1 -> xps_library_adc1x1800_10_user_data5/1, Compare To Constant6/1, Compare To Constant1/1
  delayi1/1 -> xps_library_adc1x1800_10_user_data3/1, Compare To Constant2/1, Compare To Constant4/1
  Downsamplei0/1 -> delayi0/1
  xps_library_adc1x1800_10_user_data6/1 -> conv7/1(In1)
  xps_library_adc1x1800_10_user_data4/1 -> conv6/1(In1)
  xps_library_adc1x1800_10_user_data2/1 -> conv5/1(In1)
  xps_library_adc1x1800_10_user_data0/1 -> conv4/1(In1)
  xps_library_adc1x1800_10_user_sync/1 -> sync/1
  xps_library_adc1x1800_10_user_outofrange1/1 -> outofrange1/1
  xps_library_adc1x1800_10_user_data7/1 -> conv3/1(In1)
  xps_library_adc1x1800_10_user_data5/1 -> conv2/1(In1)
  xps_library_adc1x1800_10_user_data3/1 -> conv1/1(In1)
  Downsampleq3/1 -> delayq3/1
  Downsampleq2/1 -> delayq2/1
  Downsampleq1/1 -> delayq1/1
  Downsamplei3/1 -> delayi3/1
  Downsamplei2/1 -> delayi2/1
  Downsamplei1/1 -> delayi1/1
  delayi0/1 -> xps_library_adc1x1800_10_user_data1/1, Compare To Constant/1, Compare To Constant3/1
  Downsampleq0/1 -> delayq0/1
  delayq0/1 -> xps_library_adc1x1800_10_user_data0/1, Compare To Constant11/1, Compare To Constant8/1
  Compare To Constant3/1 -> Logical Operator/1
  Compare To Constant/1 -> Logical Operator/2
  Compare To Constant4/1 -> Logical Operator5/1
  Compare To Constant2/1 -> Logical Operator5/2
  Logical Operator/1 -> xps_library_adc1x1800_10_user_outofrange1/1
  Compare To Constant6/1 -> Logical Operator1/1
  Compare To Constant1/1 -> Logical Operator1/2
  Compare To Constant7/1 -> Logical Operator6/1
  Compare To Constant5/1 -> Logical Operator6/2
  Compare To Constant11/1 -> Logical Operator2/1
  Compare To Constant8/1 -> Logical Operator2/2
  Compare To Constant12/1 -> Logical Operator7/1
  Compare To Constant10/1 -> Logical Operator7/2
  Compare To Constant14/1 -> Logical Operator3/1
  Compare To Constant9/1 -> Logical Operator3/2
  Compare To Constant15/1 -> Logical Operator8/1
  Compare To Constant13/1 -> Logical Operator8/2
  sim_sync/1 -> Downsamplesync0/1
  Downsamplesync0/1 -> delaysync0/1
  delaysync0/1 -> xps_library_adc1x1800_10_user_sync/1
  xps_library_adc1x1800_10_user_data1/1 -> conv/1(In1)
  sim_in/1 -> gain/1
  gain/1 -> bias/1
  bias/1 -> Downsamplei0/1, Downsamplei1/1, Downsamplei2/1, Downsamplei3/1, Downsampleq0/1, Downsampleq1/1, Downsampleq2/1, Downsampleq3/1
  xps_library_adc1x1800_10_user_outofrange3/1 -> outofrange3/1
  Logical Operator5/1 -> xps_library_adc1x1800_10_user_outofrange3/1
  xps_library_adc1x1800_10_user_outofrange5/1 -> outofrange5/1
  Logical Operator1/1 -> xps_library_adc1x1800_10_user_outofrange5/1
  xps_library_adc1x1800_10_user_outofrange7/1 -> outofrange7/1
  Logical Operator6/1 -> xps_library_adc1x1800_10_user_outofrange7/1
  xps_library_adc1x1800_10_user_outofrange0/1 -> outofrange0/1
  Logical Operator2/1 -> xps_library_adc1x1800_10_user_outofrange0/1
  xps_library_adc1x1800_10_user_outofrange2/1 -> outofrange2/1
  Logical Operator7/1 -> xps_library_adc1x1800_10_user_outofrange2/1
  xps_library_adc1x1800_10_user_outofrange4/1 -> outofrange4/1
  Logical Operator3/1 -> xps_library_adc1x1800_10_user_outofrange4/1
  xps_library_adc1x1800_10_user_outofrange6/1 -> outofrange6/1
  Logical Operator8/1 -> xps_library_adc1x1800_10_user_outofrange6/1
  xps_library_adc1x1800_10_user_data_valid/1 -> data_valid/1
  sim_data_valid/1 -> xps_library_adc1x1800_10_user_data_valid/1
  demux_tst_pat_en/1 -> conv_bist/1
  xps_library_adc1x1800_10_user_bist/1 -> Terminator1/1
  conv_bist/1 -> xps_library_adc1x1800_10_user_bist/1
  conv/1(Out1) -> o1/1
  conv1/1(Out1) -> o3/1
  conv2/1(Out1) -> o5/1
  conv3/1(Out1) -> o7/1
  conv4/1(Out1) -> o0/1
  conv5/1(Out1) -> o2/1
  conv6/1(Out1) -> o4/1
  conv7/1(Out1) -> o6/1
